simulink model "hopper_6dof_NED_v2_fluid_integration"  (R2026a)
settings: Solver=FixedStepAuto  StopTime=tgrid(end)  FixedStep=1e-3  RelTol=1e-5
InitFcn:
  | load('FuelPropsData.mat');
undefined symbols (not defined in the file): cg_init, dcg_dMfu_table, dcg_dMox_table, dI_dMfu_table, dI_dMox_table, ENGINE, engine_cg, engine_mass, fu_axial_damping_ratios, fu_lateral_damping_ratios, fu_mass_profile, fu_masses, fu_mdot_data, g, IN, K1flat, K2grid, MoI_init, mount_cg, OUT, ox_axial_damping_ratios, ox_lateral_damping_ratios, ox_mass_profile, ox_masses, ox_mdot_data, pressureLevels, r_leg, r_leg_1, r_leg_2, r_leg_3, r_leg_4, STRUCT, tank_r, TANKS, Target_Trajectory, tgrid, thrust_data, unom, uwndTable, VEH, vwndTable
libraries: fl_lib x43, nesl_utility x31, matrix_library x18, SimscapeFluids_lib x13, simulink x8, simulink_extras x7, slpidlib x7, dspindex x3, dspmtrx3 x3, sl_discontinuities x2, aerolibanim x1, commrandsrc3 x1
(part 7 of 7)

== system hopper_6dof_NED_v2_fluid_integration/Wind Forces/If Action Subsystem2 ==
  In1 : Inport
  Action Port : ActionPort  ActionPortLabel=else
  Display : Display
  Display1 : Display
  Latitude : Constant  Value=33.78
  Longitude : Constant  Value=84.40
  Month : Constant  Value=4
  Mux : Mux  Inputs=2
  Pressure (mb) : Constant  Value=1000
  Terminator : Terminator
  n-D Lookup Table : Lookup_n-D  NumberOfTableDimensions=4  BreakpointsForDimension1=1:12  BreakpointsForDimension2=pressureLevels  BreakpointsForDimension3=[32.5 35]  BreakpointsForDimension4=[82.5 85]  Table=uwndTable  ExtrapMethod=Clip  InternalRulePriority=Speed  RndMeth=Simplest
      settings: InputPortMap=u0,u1,u2,u3
  n-D Lookup Table1 : Lookup_n-D  NumberOfTableDimensions=4  BreakpointsForDimension1=1:12  BreakpointsForDimension2=pressureLevels  BreakpointsForDimension3=[32.5 35]  BreakpointsForDimension4=[82.5 85]  Table=vwndTable  InternalRulePriority=Speed  RndMeth=Simplest
      settings: InputPortMap=u0,u1,u2,u3
  Out1 : Outport
  wires:
  Month/1 -> n-D Lookup Table1/1, n-D Lookup Table/1
  Pressure (mb)/1 -> n-D Lookup Table1/2, n-D Lookup Table/2
  Latitude/1 -> n-D Lookup Table1/3, n-D Lookup Table/3
  In1/1 -> Terminator/1
  Longitude/1 -> n-D Lookup Table1/4, n-D Lookup Table/4
  n-D Lookup Table/1 -> Display/1, Mux/1
  n-D Lookup Table1/1 -> Display1/1, Mux/2
  Mux/1 -> Out1/1

== system hopper_6dof_NED_v2_fluid_integration/Fluid Network2/COPV/COPV Leakage ==
  Leak Rate : fl_lib/Gas/Elements/Flow Resistance (G)  delta_p_nominal=0.001 MPa  mdot_nominal=0.0000000001 kg/s  rho_nominal=0 kg/m^3  area=0.01 m^2  laminar_fraction=1e-3
  Mass & Energy Flow Rate Sensor (G)2 : fl_lib/Gas/Sensors/Flow Rate Sensor (G)  mass_flow_measure=true  volumetric_flow_measure=false  volumetric_flow_conditions=foundation.enum.volumetric_flow_conditions.actual  p_std=0.101325 MPa  T_std=20 degC  energy_flow_measure=true
  PS-Simulink Converter7 : nesl_utility/PS-Simulink Converter  PhysicalDomain=network_engine_domain  SubClassName=ps_output  LeftPortType=input  RightPortType=output  PseudoPeriodic=off  Frequencies=[]  VectorFormat=inherit  Unit=inherit  AffineConversion=off
  Pressurant Mass Leak Rate : Scope  Commented=on
      settings: ActiveDisplayYMinimum=-1  ActiveDisplayYMaximum=1
  Reservoir (G) : fl_lib/Gas/Elements/Reservoir (G)  pressure_input=false  pressure_spec=foundation.enum.pressure_spec.atmospheric  reservoir_pressure=0.101325 MPa  temperature_input=false  reservoir_temperature=293.15 K  area_A=0.01 m^2  input_error_spec=foundation.enum.input_range_error.warn
  Conn1 : PMIOPort  Side=Right
  wires:
  PS-Simulink Converter7/1 -> Pressurant Mass Leak Rate/1
  connections:
  Conn1/RConn1 -- Leak Rate/RConn1
  Leak Rate/LConn1 -- Mass & Energy Flow Rate Sensor (G)2/LConn1
  Mass & Energy Flow Rate Sensor (G)2/RConn1 -- Reservoir (G)/LConn1
  Mass & Energy Flow Rate Sensor (G)2/RConn2 -- PS-Simulink Converter7/LConn1

== system hopper_6dof_NED_v2_fluid_integration/Fluid Network2/Physical Combustion Chamber1/Ox Tank PT + Initial Conditions2 ==
  Initial OT Pressure : InitialCondition  Value=500
  PS-Simulink Converter3 : nesl_utility/PS-Simulink Converter  PhysicalDomain=network_engine_domain  SubClassName=ps_output  LeftPortType=input  RightPortType=output  PseudoPeriodic=off  Frequencies=[]  VectorFormat=inherit  Unit=inherit  AffineConversion=off
  Pa to psi : Gain  Gain=0.000145038
  Pressure & Temperature Sensor (TL) : fl_lib/Thermal Liquid/Sensors/Pressure & Temperature Sensor (TL)  reference=foundation.enum.MeasurementReference.absolute  pressure=true  pressure_spec=foundation.enum.PressureMeasementSpec.Gauge  temperature=false
  fuel line : PMIOPort  Side=Left
  Out1 : Outport
  wires:
  Initial OT Pressure/1 -> Out1/1
  Pa to psi/1 -> Initial OT Pressure/1
  PS-Simulink Converter3/1 -> Pa to psi/1
  connections:
  PS-Simulink Converter3/LConn1 -- Pressure & Temperature Sensor (TL)/RConn1
  Pressure & Temperature Sensor (TL)/LConn1 -- fuel line/RConn1

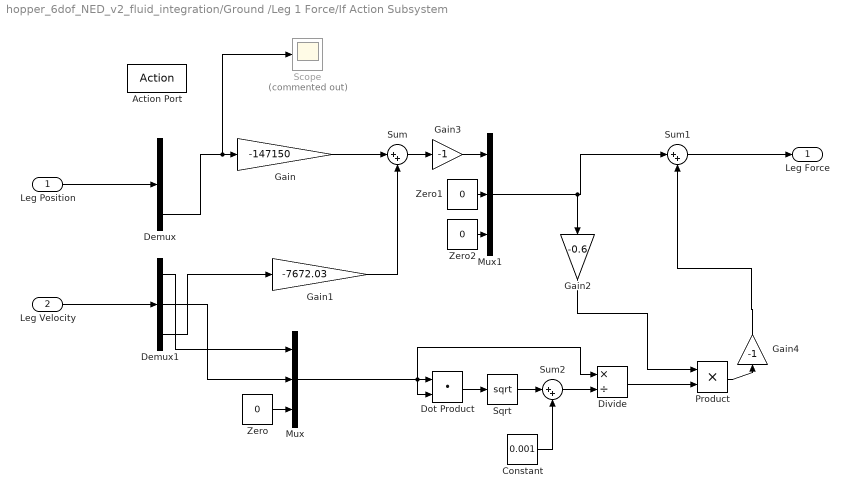
== system hopper_6dof_NED_v2_fluid_integration/Ground /Leg 1 Force/If Action Subsystem ==
  Leg Position : Inport
  Leg Velocity : Inport  Port=2
  Action Port : ActionPort  ActionPortLabel=|
      | if(u1 > -0.001 
      | )
  Constant : Constant  Value=0.001
  Demux : Demux  Outputs=3
  Demux1 : Demux  Outputs=3
  Divide : Product  Inputs=*/
  Dot Product : DotProduct  OutDataTypeStr=Inherit: Inherit via internal rule
  Gain : Gain  Gain=-147150
  Gain1 : Gain  Gain=-7672.03
  Gain2 : Gain  Gain=-0.6
  Gain3 : Gain  Gain=-1
  Gain4 : Gain  Gain=-1
  Mux : Mux  Inputs=3
  Mux1 : Mux  Inputs=3
  Product : Product
  Scope : Scope  Commented=on
      settings: ActiveDisplayYMinimum=-1  ActiveDisplayYMaximum=1  DataLoggingVariableName=ScopeData69
  Sqrt : Sqrt
  Sum : Sum  Inputs=|++
  Sum1 : Sum  Inputs=|++
  Sum2 : Sum  Inputs=|++
  Zero : Constant  Value=0  OutDataTypeStr=Inherit: Inherit via back propagation
  Zero1 : Constant  Value=0  OutDataTypeStr=Inherit: Inherit via back propagation
  Zero2 : Constant  Value=0  OutDataTypeStr=Inherit: Inherit via back propagation
  Leg Force : Outport
  wires:
  Leg Position/1 -> Demux/1
  Leg Velocity/1 -> Demux1/1
  Gain/1 -> Sum/1
  Gain1/1 -> Sum/2
  Demux1/3 -> Gain1/1
  Demux1/2 -> Mux/2
  Demux1/1 -> Mux/1
  Mux/1 -> Dot Product/2, Dot Product/1, Divide/1
  Dot Product/1 -> Sqrt/1
  Divide/1 -> Product/2
  Gain2/1 -> Product/1
  Product/1 -> Gain4/1
  Sum1/1 -> Leg Force/1
  Sqrt/1 -> Sum2/1
  Sum2/1 -> Divide/2
  Constant/1 -> Sum2/2
  Sum/1 -> Gain3/1
  Zero1/1 -> Mux1/2
  Zero2/1 -> Mux1/3
  Mux1/1 -> Sum1/1, Gain2/1
  Demux/3 -> Scope/1, Gain/1
  Zero/1 -> Mux/3
  Gain3/1 -> Mux1/1
  Gain4/1 -> Sum1/2

== system hopper_6dof_NED_v2_fluid_integration/Ground /Leg 1 Force/If Action Subsystem1 ==
  Action Port : ActionPort  ActionPortLabel=else
  Constant : Constant  Value=[0 0 0]
  Out1 : Outport
  wires:
  Constant/1 -> Out1/1

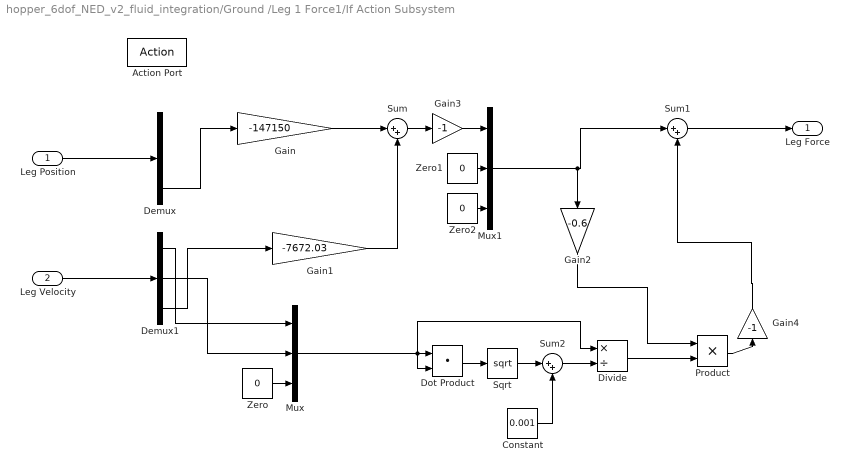
== system hopper_6dof_NED_v2_fluid_integration/Ground /Leg 1 Force1/If Action Subsystem ==
  Leg Position : Inport
  Leg Velocity : Inport  Port=2
  Action Port : ActionPort  ActionPortLabel=|
      | if(u1 > -0.001 
      | )
  Constant : Constant  Value=0.001
  Demux : Demux  Outputs=3
  Demux1 : Demux  Outputs=3
  Divide : Product  Inputs=*/
  Dot Product : DotProduct  OutDataTypeStr=Inherit: Inherit via internal rule
  Gain : Gain  Gain=-147150
  Gain1 : Gain  Gain=-7672.03
  Gain2 : Gain  Gain=-0.6
  Gain3 : Gain  Gain=-1
  Gain4 : Gain  Gain=-1
  Mux : Mux  Inputs=3
  Mux1 : Mux  Inputs=3
  Product : Product
  Sqrt : Sqrt
  Sum : Sum  Inputs=|++
  Sum1 : Sum  Inputs=|++
  Sum2 : Sum  Inputs=|++
  Zero : Constant  Value=0  OutDataTypeStr=Inherit: Inherit via back propagation
  Zero1 : Constant  Value=0  OutDataTypeStr=Inherit: Inherit via back propagation
  Zero2 : Constant  Value=0  OutDataTypeStr=Inherit: Inherit via back propagation
  Leg Force : Outport
  wires:
  Leg Position/1 -> Demux/1
  Leg Velocity/1 -> Demux1/1
  Gain/1 -> Sum/1
  Gain1/1 -> Sum/2
  Demux1/3 -> Gain1/1
  Demux1/2 -> Mux/2
  Demux1/1 -> Mux/1
  Mux/1 -> Dot Product/2, Dot Product/1, Divide/1
  Dot Product/1 -> Sqrt/1
  Divide/1 -> Product/2
  Gain2/1 -> Product/1
  Product/1 -> Gain4/1
  Sum1/1 -> Leg Force/1
  Sqrt/1 -> Sum2/1
  Sum2/1 -> Divide/2
  Constant/1 -> Sum2/2
  Sum/1 -> Gain3/1
  Zero1/1 -> Mux1/2
  Zero2/1 -> Mux1/3
  Mux1/1 -> Sum1/1, Gain2/1
  Demux/3 -> Gain/1
  Zero/1 -> Mux/3
  Gain3/1 -> Mux1/1
  Gain4/1 -> Sum1/2

== system hopper_6dof_NED_v2_fluid_integration/Ground /Leg 1 Force1/If Action Subsystem1 ==
  Action Port : ActionPort  ActionPortLabel=else
  Constant : Constant  Value=[0 0 0]
  Out1 : Outport
  wires:
  Constant/1 -> Out1/1

== system hopper_6dof_NED_v2_fluid_integration/Ground /Leg 1 Force2/If Action Subsystem ==
  Leg Position : Inport
  Leg Velocity : Inport  Port=2
  Action Port : ActionPort  ActionPortLabel=|
      | if(u1 > -0.001 
      | )
  Constant : Constant  Value=0.001
  Demux : Demux  Outputs=3
  Demux1 : Demux  Outputs=3
  Divide : Product  Inputs=*/
  Dot Product : DotProduct  OutDataTypeStr=Inherit: Inherit via internal rule
  Gain : Gain  Gain=-147150
  Gain1 : Gain  Gain=-7672.03
  Gain2 : Gain  Gain=-0.6
  Gain3 : Gain  Gain=-1
  Gain4 : Gain  Gain=-1
  Mux : Mux  Inputs=3
  Mux1 : Mux  Inputs=3
  Product : Product
  Sqrt : Sqrt
  Sum : Sum  Inputs=|++
  Sum1 : Sum  Inputs=|++
  Sum2 : Sum  Inputs=|++
  Zero : Constant  Value=0  OutDataTypeStr=Inherit: Inherit via back propagation
  Zero1 : Constant  Value=0  OutDataTypeStr=Inherit: Inherit via back propagation
  Zero2 : Constant  Value=0  OutDataTypeStr=Inherit: Inherit via back propagation
  Leg Force : Outport
  wires:
  Leg Position/1 -> Demux/1
  Leg Velocity/1 -> Demux1/1
  Gain/1 -> Sum/1
  Gain1/1 -> Sum/2
  Demux1/3 -> Gain1/1
  Demux1/2 -> Mux/2
  Demux1/1 -> Mux/1
  Mux/1 -> Dot Product/2, Dot Product/1, Divide/1
  Dot Product/1 -> Sqrt/1
  Divide/1 -> Product/2
  Gain2/1 -> Product/1
  Product/1 -> Gain4/1
  Sum1/1 -> Leg Force/1
  Sqrt/1 -> Sum2/1
  Sum2/1 -> Divide/2
  Constant/1 -> Sum2/2
  Sum/1 -> Gain3/1
  Zero1/1 -> Mux1/2
  Zero2/1 -> Mux1/3
  Mux1/1 -> Sum1/1, Gain2/1
  Demux/3 -> Gain/1
  Zero/1 -> Mux/3
  Gain3/1 -> Mux1/1
  Gain4/1 -> Sum1/2

== system hopper_6dof_NED_v2_fluid_integration/Ground /Leg 1 Force2/If Action Subsystem1 ==
  Action Port : ActionPort  ActionPortLabel=else
  Constant : Constant  Value=[0 0 0]
  Out1 : Outport
  wires:
  Constant/1 -> Out1/1

== system hopper_6dof_NED_v2_fluid_integration/Ground /Leg 1 Force3/If Action Subsystem ==
  Leg Position : Inport
  Leg Velocity : Inport  Port=2
  Action Port : ActionPort  ActionPortLabel=|
      | if(u1 > -0.001 
      | )
  Constant : Constant  Value=0.001
  Demux : Demux  Outputs=3
  Demux1 : Demux  Outputs=3
  Divide : Product  Inputs=*/
  Dot Product : DotProduct  OutDataTypeStr=Inherit: Inherit via internal rule
  Gain : Gain  Gain=-147150
  Gain1 : Gain  Gain=-7672.03
  Gain2 : Gain  Gain=-0.6
  Gain3 : Gain  Gain=-1
  Gain4 : Gain  Gain=-1
  Mux : Mux  Inputs=3
  Mux1 : Mux  Inputs=3
  Product : Product
  Sqrt : Sqrt
  Sum : Sum  Inputs=|++
  Sum1 : Sum  Inputs=|++
  Sum2 : Sum  Inputs=|++
  Zero : Constant  Value=0  OutDataTypeStr=Inherit: Inherit via back propagation
  Zero1 : Constant  Value=0  OutDataTypeStr=Inherit: Inherit via back propagation
  Zero2 : Constant  Value=0  OutDataTypeStr=Inherit: Inherit via back propagation
  Leg Force : Outport
  wires:
  Leg Position/1 -> Demux/1
  Leg Velocity/1 -> Demux1/1
  Gain/1 -> Sum/1
  Gain1/1 -> Sum/2
  Demux1/3 -> Gain1/1
  Demux1/2 -> Mux/2
  Demux1/1 -> Mux/1
  Mux/1 -> Dot Product/2, Dot Product/1, Divide/1
  Dot Product/1 -> Sqrt/1
  Divide/1 -> Product/2
  Gain2/1 -> Product/1
  Product/1 -> Gain4/1
  Sum1/1 -> Leg Force/1
  Sqrt/1 -> Sum2/1
  Sum2/1 -> Divide/2
  Constant/1 -> Sum2/2
  Sum/1 -> Gain3/1
  Zero1/1 -> Mux1/2
  Zero2/1 -> Mux1/3
  Mux1/1 -> Sum1/1, Gain2/1
  Demux/3 -> Gain/1
  Zero/1 -> Mux/3
  Gain3/1 -> Mux1/1
  Gain4/1 -> Sum1/2

== system hopper_6dof_NED_v2_fluid_integration/Ground /Leg 1 Force3/If Action Subsystem1 ==
  Action Port : ActionPort  ActionPortLabel=else
  Constant : Constant  Value=[0 0 0]
  Out1 : Outport
  wires:
  Constant/1 -> Out1/1

== matlab function hopper_6dof_NED_v2_fluid_integration/Slosh/Oxidizer Yaw Force/MATLAB Function ==
  data: ox_yaw_accel input; accel_term output; ox_lateral_pendulum_l input
function accel_term = fcn(ox_yaw_accel, ox_lateral_pendulum_l)

accel_term = -ox_yaw_accel / ox_lateral_pendulum_l;

end

== matlab function hopper_6dof_NED_v2_fluid_integration/Slosh/Oxidizer Yaw Force/MATLAB Function1 ==
  data: ox_yaw_phi input; ang_term output; ox_lateral_natural_freq input
function ang_term = fcn(ox_yaw_phi, ox_lateral_natural_freq)

ang_term = -ox_lateral_natural_freq^2 * ox_yaw_phi;

end

== matlab function hopper_6dof_NED_v2_fluid_integration/Slosh/Oxidizer Yaw Force/MATLAB Function2 ==
  data: ox_yaw_phi_dot input; velo_term output; ox_lateral_natural_freq input; ox_lateral_damping input
function velo_term = fcn(ox_yaw_phi_dot, ox_lateral_natural_freq,ox_lateral_damping)

velo_term = -2 * ox_lateral_damping * ox_lateral_natural_freq * ox_yaw_phi_dot;
end

== matlab function hopper_6dof_NED_v2_fluid_integration/Slosh/Oxidizer Yaw Force/MATLAB Function3 ==
  data: ox_yaw_phi_ddot input; ox_yaw_f output; ox_lateral_slosh_mass input; ox_lateral_pendulum_l input
function ox_yaw_f = fcn(ox_yaw_phi_ddot, ox_lateral_slosh_mass, ox_lateral_pendulum_l)
% Force of the pendulum on the tank, beyond the rigid propellant already in
% the vehicle mass: -m1 * y_ddot, y = l*phi the body-frame bob displacement
% (phi_ddot = -a/l - w^2 phi - 2 zeta w phi_dot). Sign was +m1*y_ddot,
% which added m1 to the lateral inertia instead of removing it.
ox_yaw_f = -ox_lateral_slosh_mass * ox_lateral_pendulum_l * ox_yaw_phi_ddot;
end

== matlab function hopper_6dof_NED_v2_fluid_integration/Slosh/Oxidizer Axial Force/MATLAB Function ==
  data: ox_axial_accel input; accel_term output; ox_axial_pendulum_l input
function accel_term = fcn(ox_axial_accel, ox_axial_pendulum_l)

accel_term = -ox_axial_accel / ox_axial_pendulum_l;

end

== matlab function hopper_6dof_NED_v2_fluid_integration/Slosh/Oxidizer Axial Force/MATLAB Function1 ==
  data: ox_axial_phi input; ang_term output; ox_axial_natural_freq input
function ang_term = fcn(ox_axial_phi, ox_axial_natural_freq)

ang_term = -ox_axial_natural_freq^2 * ox_axial_phi;

end

== matlab function hopper_6dof_NED_v2_fluid_integration/Slosh/Oxidizer Axial Force/MATLAB Function2 ==
  data: ox_axial_phi_dot input; velo_term output; ox_axial_natural_freq input; ox_axial_damping input
function velo_term = fcn(ox_axial_phi_dot, ox_axial_natural_freq,ox_axial_damping)

velo_term = -2 * ox_axial_damping * ox_axial_natural_freq * ox_axial_phi_dot;
end

== matlab function hopper_6dof_NED_v2_fluid_integration/Slosh/Oxidizer Axial Force/MATLAB Function3 ==
  data: ox_axial_phi_ddot input; ox_axial_f output; ox_axial_slosh_mass input; ox_axial_pendulum_l input
function ox_axial_f = fcn(ox_axial_phi_ddot, ox_axial_slosh_mass, ox_axial_pendulum_l)
% Force of the pendulum on the tank, beyond the rigid propellant already in
% the vehicle mass: -m1 * y_ddot, y = l*phi the body-frame bob displacement
% (phi_ddot = -a/l - w^2 phi - 2 zeta w phi_dot). Sign was +m1*y_ddot,
% which added m1 to the lateral inertia instead of removing it.
ox_axial_f = -ox_axial_slosh_mass * ox_axial_pendulum_l * ox_axial_phi_ddot;
end

== matlab function hopper_6dof_NED_v2_fluid_integration/Slosh/Fuel Axial Force/MATLAB Function ==
  data: fu_axial_accel input; accel_term output; fu_axial_pendulum_l input
function accel_term = fcn(fu_axial_accel, fu_axial_pendulum_l)

accel_term = -fu_axial_accel / fu_axial_pendulum_l;

end

== matlab function hopper_6dof_NED_v2_fluid_integration/Slosh/Fuel Axial Force/MATLAB Function1 ==
  data: fu_axial_phi input; ang_term output; fu_axial_natural_freq input
function ang_term = fcn(fu_axial_phi, fu_axial_natural_freq)

ang_term = -fu_axial_natural_freq^2 * fu_axial_phi;

end

== matlab function hopper_6dof_NED_v2_fluid_integration/Slosh/Fuel Axial Force/MATLAB Function2 ==
  data: fu_axial_phi_dot input; velo_term output; fu_axial_natural_freq input; fu_axial_damping input
function velo_term = fcn(fu_axial_phi_dot, fu_axial_natural_freq,fu_axial_damping)

velo_term = -2 * fu_axial_damping * fu_axial_natural_freq * fu_axial_phi_dot;
end

== matlab function hopper_6dof_NED_v2_fluid_integration/Slosh/Fuel Axial Force/MATLAB Function3 ==
  data: fu_axial_phi_ddot input; fu_axial_f output; fu_axial_slosh_mass input; fu_axial_pendulum_l input
function fu_axial_f = fcn(fu_axial_phi_ddot, fu_axial_slosh_mass, fu_axial_pendulum_l)
% Force of the pendulum on the tank, beyond the rigid propellant already in
% the vehicle mass: -m1 * y_ddot, y = l*phi the body-frame bob displacement
% (phi_ddot = -a/l - w^2 phi - 2 zeta w phi_dot). Sign was +m1*y_ddot,
% which added m1 to the lateral inertia instead of removing it.
fu_axial_f = -fu_axial_slosh_mass * fu_axial_pendulum_l * fu_axial_phi_ddot;
end

== matlab function hopper_6dof_NED_v2_fluid_integration/Slosh/Fuel Yaw Force/MATLAB Function ==
  data: fu_pitch_accel input; accel_term output; fu_lateral_pendulum_l input
function accel_term = fcn(fu_pitch_accel, fu_lateral_pendulum_l)

accel_term = -fu_pitch_accel / fu_lateral_pendulum_l;

end

== matlab function hopper_6dof_NED_v2_fluid_integration/Slosh/Fuel Yaw Force/MATLAB Function1 ==
  data: fu_pitch_phi input; ang_term output; fu_lateral_natural_freq input
function ang_term = fcn(fu_pitch_phi, fu_lateral_natural_freq)

ang_term = -fu_lateral_natural_freq^2 * fu_pitch_phi;

end

== matlab function hopper_6dof_NED_v2_fluid_integration/Slosh/Fuel Yaw Force/MATLAB Function2 ==
  data: fu_pitch_phi_dot input; velo_term output; fu_lateral_natural_freq input; fu_lateral_damping input
function velo_term = fcn(fu_pitch_phi_dot, fu_lateral_natural_freq,fu_lateral_damping)

velo_term = -2 * fu_lateral_damping * fu_lateral_natural_freq * fu_pitch_phi_dot;
end

== matlab function hopper_6dof_NED_v2_fluid_integration/Slosh/Fuel Yaw Force/MATLAB Function3 ==
  data: fu_pitch_phi_ddot input; fu_pitch_f output; fu_lateral_slosh_mass input; fu_lateral_pendulum_l input
function fu_pitch_f = fcn(fu_pitch_phi_ddot, fu_lateral_slosh_mass, fu_lateral_pendulum_l)
% Force of the pendulum on the tank, beyond the rigid propellant already in
% the vehicle mass: -m1 * y_ddot, y = l*phi the body-frame bob displacement
% (phi_ddot = -a/l - w^2 phi - 2 zeta w phi_dot). Sign was +m1*y_ddot,
% which added m1 to the lateral inertia instead of removing it.
fu_pitch_f = -fu_lateral_slosh_mass * fu_lateral_pendulum_l * fu_pitch_phi_ddot;
end

== matlab function hopper_6dof_NED_v2_fluid_integration/Slosh/Fuel Pitch Force/MATLAB Function ==
  data: fu_yaw_accel input; accel_term output; fu_lateral_pendulum_l input
function accel_term = fcn(fu_yaw_accel, fu_lateral_pendulum_l)

accel_term = -fu_yaw_accel / fu_lateral_pendulum_l;

end

== matlab function hopper_6dof_NED_v2_fluid_integration/Slosh/MATLAB Function ==
  data: ox_lateral_natural_freq output; ox_axial_natural_freq output; ox_mass input; ox_lateral_slosh_mass output; ox_axial_slosh_mass output; ox_lateral_pendulum_l output; ox_aeff input; ox_axial_pendulum_l output; ox_lateral_damping output; ox_axial_damping output; tank_r input; ox_lateral_damping input; ox_axial_damping input
function [ox_lateral_natural_freq, ox_axial_natural_freq, ox_lateral_slosh_mass,ox_axial_slosh_mass, ox_lateral_pendulum_l, ox_axial_pendulum_l, ox_lateral_damping, ox_axial_damping]  = slosh_parameters(ox_mass, ox_aeff, tank_r, ox_lateral_damping, ox_axial_damping)

% Flat-bottomed cylindrical tank, linear slosh (NASA SP-106 / Dodge 2000;
% lateral values checked against SLOSH-ML, lgst-lab/slosh_ml).
zeta = 1.841;    % 1st root of J1' (1st lateral mode)
eps01 = 3.8317;  % 1st root of J1 (1st axisymmetric mode)
ox_density = 1141;   % kg/m^3
geff = norm(ox_aeff) + 0.001;

if ox_mass > 0.001
   h_ox_fluid = (ox_mass / ox_density) / (pi * tank_r^2);

   % Lateral mode: omega^2 = (g*xi/R) * tanh(xi*h/R)
    ox_lateral_natural_freq = sqrt(zeta * geff / tank_r * tanh(zeta * h_ox_fluid / tank_r));
    ox_lateral_slosh_mass = ox_mass * (2 * tank_r * tanh(zeta * h_ox_fluid / tank_r)) / (zeta * (zeta^2 - 1) * h_ox_fluid);
    ox_lateral_pendulum_l = tank_r / (zeta * tanh(zeta * h_ox_fluid / tank_r));   % = geff / omega^2

    % Axisymmetric (m = 0) mode: omega^2 = (g*eps01/R) * tanh(eps01*h/R).
    % Volume is conserved and the mode is axisymmetric, so to first order
    % it puts no net force or moment on the tank: its equivalent mechanical
    % mass is zero. The oscillator is kept (frequency/damping) but couples
    % no force or roll torque into the vehicle.
    ox_axial_natural_freq = sqrt(eps01 * geff / tank_r * tanh(eps01 * h_ox_fluid / tank_r));
    ox_axial_slosh_mass = 0;
    ox_axial_pendulum_l = geff / ox_axial_natural_freq^2;
else
   h_ox_fluid = 0;
   ox_lateral_natural_freq = 0;
   ox_axial_natural_freq = 0;
   ox_lateral_slosh_mass = 0;
   ox_axial_slosh_mass = 0;
   ox_lateral_pendulum_l = 1;
   ox_axial_pendulum_l = 1;
end

end

== matlab function hopper_6dof_NED_v2_fluid_integration/Slosh/Fuel Pitch Force/MATLAB Function1 ==
  data: fu_yaw_phi input; ang_term output; fu_lateral_natural_freq input
function ang_term = fcn(fu_yaw_phi, fu_lateral_natural_freq)

ang_term = -fu_lateral_natural_freq^2 * fu_yaw_phi;

end

== matlab function hopper_6dof_NED_v2_fluid_integration/Slosh/Fuel Pitch Force/MATLAB Function2 ==
  data: fu_yaw_phi_dot input; velo_term output; fu_lateral_natural_freq input; fu_lateral_damping input
function velo_term = fcn(fu_yaw_phi_dot, fu_lateral_natural_freq, fu_lateral_damping)

velo_term = -2 * fu_lateral_damping * fu_lateral_natural_freq * fu_yaw_phi_dot;
end

== matlab function hopper_6dof_NED_v2_fluid_integration/Slosh/Fuel Pitch Force/MATLAB Function3 ==
  data: fu_yaw_phi_ddot input; fu_yaw_f output; fu_lateral_slosh_mass input; fu_lateral_pendulum_l input
function fu_yaw_f = fcn(fu_yaw_phi_ddot, fu_lateral_slosh_mass, fu_lateral_pendulum_l)
% Force of the pendulum on the tank, beyond the rigid propellant already in
% the vehicle mass: -m1 * y_ddot, y = l*phi the body-frame bob displacement
% (phi_ddot = -a/l - w^2 phi - 2 zeta w phi_dot). Sign was +m1*y_ddot,
% which added m1 to the lateral inertia instead of removing it.
fu_yaw_f = -fu_lateral_slosh_mass * fu_lateral_pendulum_l * fu_yaw_phi_ddot;
end

== matlab function hopper_6dof_NED_v2_fluid_integration/CG // MOI Script v3/MATLAB Function ==
  data: r_ox input; I_m_ox output
function I_m_ox = fcn(r_ox)
% Slosh point-mass inertia contribution. The base MOI (cg_moi_init /
% dI_dMox LUT) already carries all the propellant as a rigid body, and
% the slosh pendulum dynamics reach the vehicle through Slosh_F / Slosh_M,
% so adding the slosh masses again here double counts them (and r_ox is
% measured from the vehicle datum, not the CG). Contribution removed;
% output kept so the block interface is unchanged.
% (Previous parallel-axis tensor also had sign errors in its products
% of inertia and was not symmetric.)
I_m_ox = zeros(3) * r_ox(1);

== matlab function hopper_6dof_NED_v2_fluid_integration/CG // MOI Script v3/MATLAB Function1 ==
  data: r_fu input; I_m_fu output
function I_m_fu = fcn(r_fu)
% Slosh point-mass inertia contribution. The base MOI (cg_moi_init /
% dI_dMfu LUT) already carries all the propellant as a rigid body, and
% the slosh pendulum dynamics reach the vehicle through Slosh_F / Slosh_M,
% so adding the slosh masses again here double counts them (and r_fu is
% measured from the vehicle datum, not the CG). Contribution removed;
% output kept so the block interface is unchanged.
% (Previous parallel-axis tensor also had sign errors in its products
% of inertia and was not symmetric.)
I_m_fu = zeros(3) * r_fu(1);

== matlab function hopper_6dof_NED_v2_fluid_integration/Slosh/Oxidizer Axial Force/MATLAB Function4 ==
  data: x_omega_dot input; x_slosh_torque output; ox_axial_slosh_mass input; ox_axial_pendulum_l input; slosh_angular_accel input
function x_slosh_torque = fcn(x_omega_dot, ox_axial_slosh_mass, ox_axial_pendulum_l, slosh_angular_accel)
% Per-pendulum torque removed. A pendulum analog (SP-106, Dodge 2000,
% SLOSH-ML) is a point mass on a frictionless hinge: it has no rotational
% inertia of its own and transmits no moment through the hinge. The old
% -m*l^2*(omega_dot - phi_ddot) term added a fictitious inertia m*l^2 and a
% hinge moment. The liquid rigid-body inertia (the analog's I0) is carried
% by the CG/MOI tables. Inputs kept for the
% subsystem interface.
x_slosh_torque = 0 * x_omega_dot;
end

== matlab function hopper_6dof_NED_v2_fluid_integration/Slosh/Fuel Axial Force/MATLAB Function4 ==
  data: x_omega_dot input; x_slosh_torque output; fu_axial_slosh_mass input; fu_axial_pendulum_l input; slosh_angular_accel input
function x_slosh_torque = fcn(x_omega_dot, fu_axial_slosh_mass, fu_axial_pendulum_l, slosh_angular_accel)
% Per-pendulum torque removed. A pendulum analog (SP-106, Dodge 2000,
% SLOSH-ML) is a point mass on a frictionless hinge: it has no rotational
% inertia of its own and transmits no moment through the hinge. The old
% -m*l^2*(omega_dot - phi_ddot) term added a fictitious inertia m*l^2 and a
% hinge moment. The liquid rigid-body inertia (the analog's I0) is carried
% by the CG/MOI tables. Inputs kept for the
% subsystem interface.
x_slosh_torque = 0 * x_omega_dot;
end

== matlab function hopper_6dof_NED_v2_fluid_integration/Slosh/Oxidizer Yaw Force/MATLAB Function4 ==
  data: y_omega_dot input; y_slosh_torque output; ox_lateral_slosh_mass input; ox_lateral_pendulum_l input; slosh_angular_accel input
function y_slosh_torque = fcn(y_omega_dot, ox_lateral_slosh_mass, ox_lateral_pendulum_l, slosh_angular_accel)
% Per-pendulum torque removed. A pendulum analog (SP-106, Dodge 2000,
% SLOSH-ML) is a point mass on a frictionless hinge: it has no rotational
% inertia of its own and transmits no moment through the hinge. The old
% -m*l^2*(omega_dot - phi_ddot) term added a fictitious inertia m*l^2 and a
% hinge moment. The liquid rigid-body inertia (the analog's I0) is carried
% by the CG/MOI tables. Inputs kept for the
% subsystem interface.
y_slosh_torque = 0 * y_omega_dot;
end

== matlab function hopper_6dof_NED_v2_fluid_integration/Slosh/Fuel Yaw Force/MATLAB Function4 ==
  data: y_omega_dot input; y_slosh_torque output; fu_lateral_slosh_mass input; fu_lateral_pendulum_l input; slosh_angular_accel input
function y_slosh_torque = fcn(y_omega_dot, fu_lateral_slosh_mass, fu_lateral_pendulum_l, slosh_angular_accel)
% Per-pendulum torque removed. A pendulum analog (SP-106, Dodge 2000,
% SLOSH-ML) is a point mass on a frictionless hinge: it has no rotational
% inertia of its own and transmits no moment through the hinge. The old
% -m*l^2*(omega_dot - phi_ddot) term added a fictitious inertia m*l^2 and a
% hinge moment. The liquid rigid-body inertia (the analog's I0) is carried
% by the CG/MOI tables. Inputs kept for the
% subsystem interface.
y_slosh_torque = 0 * y_omega_dot;
end

== matlab function hopper_6dof_NED_v2_fluid_integration/Slosh/Oxidizer Pitch Force/MATLAB Function4 ==
  data: z_omega_dot input; z_slosh_torque output; ox_lateral_slosh_mass input; ox_lateral_pendulum_l input; slosh_angular_accel input
function z_slosh_torque = fcn(z_omega_dot, ox_lateral_slosh_mass, ox_lateral_pendulum_l, slosh_angular_accel)
% Per-pendulum torque removed. A pendulum analog (SP-106, Dodge 2000,
% SLOSH-ML) is a point mass on a frictionless hinge: it has no rotational
% inertia of its own and transmits no moment through the hinge. The old
% -m*l^2*(omega_dot - phi_ddot) term added a fictitious inertia m*l^2 and a
% hinge moment. The liquid rigid-body inertia (the analog's I0) is carried
% by the CG/MOI tables. Inputs kept for the
% subsystem interface.
z_slosh_torque = 0 * z_omega_dot;
end

== matlab function hopper_6dof_NED_v2_fluid_integration/Slosh/Fuel Pitch Force/MATLAB Function4 ==
  data: z_omega_dot input; z_slosh_torque output; fu_lateral_slosh_mass input; fu_lateral_pendulum_l input; slosh_angular_accel input
function z_slosh_torque = fcn(z_omega_dot, fu_lateral_slosh_mass, fu_lateral_pendulum_l, slosh_angular_accel)
% Per-pendulum torque removed. A pendulum analog (SP-106, Dodge 2000,
% SLOSH-ML) is a point mass on a frictionless hinge: it has no rotational
% inertia of its own and transmits no moment through the hinge. The old
% -m*l^2*(omega_dot - phi_ddot) term added a fictitious inertia m*l^2 and a
% hinge moment. The liquid rigid-body inertia (the analog's I0) is carried
% by the CG/MOI tables. Inputs kept for the
% subsystem interface.
z_slosh_torque = 0 * z_omega_dot;
end

== matlab function hopper_6dof_NED_v2_fluid_integration/CG // MOI Script v3/MATLAB Function2 ==
  data: delta_y input; rot_mat output; delta_z input
function rot_mat = fcn(delta_y, delta_z)

rot_mat = [0 -delta_z delta_y;
           delta_z 0 0;
           -delta_y 0 0];

== matlab function hopper_6dof_NED_v2_fluid_integration/Slosh/Ox Slosh Mass Location ==
  data: r_floor input; r_bob output; ox_mass input; tank_r input
function r_bob = fcn(r_floor, ox_mass, tank_r)
% Rest position of the 1st lateral pendulum bob (= spring-mass location),
% flat-bottom cylinder, NASA SP-106 / Dodge 2000:
%   H1 = h - (2R/xi) tanh(xi h / 2R)  above the tank floor,
%   hinge = H1 + L1,  L1 = R / (xi tanh(xi h / R)).
% Matches SLOSH-ML (validation/slosh_ml/compareSloshML.m) to < 2 mm.
% The slosh force is applied here, not at the hinge: the propellant
% (bob included) is already a rigid body in the CG/MOI tables, so the
% pendulum correction is -m1*y_ddot at the bob rest point plus the
% offset moment -m1*y x f (Slosh offset moment blocks); together these
% equal the rod force acting at the hinge.
% r_floor is in the Slosh frame (datum x negated).
xi = 1.841;
ox_density = 1141;   % kg/m^3
h = (ox_mass / ox_density) / (pi * tank_r^2);
H1 = h - (2 * tank_r / xi) * tanh(xi * h / (2 * tank_r));
r_bob = r_floor;
r_bob(1) = r_floor(1) - H1;

== matlab function hopper_6dof_NED_v2_fluid_integration/Slosh/Fu Slosh Mass Location ==
  data: r_floor input; r_bob output; fu_mass input; tank_r input
function r_bob = fcn(r_floor, fu_mass, tank_r)
% Rest position of the 1st lateral pendulum bob (= spring-mass location),
% flat-bottom cylinder, NASA SP-106 / Dodge 2000:
%   H1 = h - (2R/xi) tanh(xi h / 2R)  above the tank floor,
%   hinge = H1 + L1,  L1 = R / (xi tanh(xi h / R)).
% Matches SLOSH-ML (validation/slosh_ml/compareSloshML.m) to < 2 mm.
% The slosh force is applied here, not at the hinge: the propellant
% (bob included) is already a rigid body in the CG/MOI tables, so the
% pendulum correction is -m1*y_ddot at the bob rest point plus the
% offset moment -m1*y x f (Slosh offset moment blocks); together these
% equal the rod force acting at the hinge.
% r_floor is in the Slosh frame (datum x negated).
xi = 1.841;
fu_density = 800;   % kg/m^3
h = (fu_mass / fu_density) / (pi * tank_r^2);
H1 = h - (2 * tank_r / xi) * tanh(xi * h / (2 * tank_r));
r_bob = r_floor;
r_bob(1) = r_floor(1) - H1;

== matlab function hopper_6dof_NED_v2_fluid_integration/Slosh/Ox Slosh Offset Moment ==
  data: ox_slosh_pos input; M output; ox_slosh_mass input; ox_a_eff input
function M = fcn(ox_slosh_pos, ox_slosh_mass, ox_a_eff)
% Moment about the CG from the slosh mass displaced by y from its rest
% point, under the specific force f at the tank: -m1 * y x f. With the
% -m1*y_ddot force at the rest point this is the first-order pendulum
% load (rod force at the hinge). Replaces the slosh CG shift in
% CG // MOI Script v3, which divided by the propellant mass instead of
% the vehicle mass, had the lateral sign reversed, and was delayed.
M = reshape(-cross(ox_slosh_mass(:) .* ox_slosh_pos(:), ox_a_eff(:)), size(ox_a_eff));

== matlab function hopper_6dof_NED_v2_fluid_integration/Slosh/Fu Slosh Offset Moment ==
  data: fu_slosh_pos input; M output; fu_slosh_mass input; fu_a_eff input
function M = fcn(fu_slosh_pos, fu_slosh_mass, fu_a_eff)
% Moment about the CG from the slosh mass displaced by y from its rest
% point, under the specific force f at the tank: -m1 * y x f. With the
% -m1*y_ddot force at the rest point this is the first-order pendulum
% load (rod force at the hinge). Replaces the slosh CG shift in
% CG // MOI Script v3, which divided by the propellant mass instead of
% the vehicle mass, had the lateral sign reversed, and was delayed.
M = reshape(-cross(fu_slosh_mass(:) .* fu_slosh_pos(:), fu_a_eff(:)), size(fu_a_eff));

== matlab function hopper_6dof_NED_v2_fluid_integration/CG // MOI Script v3/Slosh Diagnostics ==
  data: cg input; cg_with_slosh output; MOI input; ox_slosh_pos input; fu_slosh_pos input; ox_slosh_mass input; fu_slosh_mass input; m_ox input; m_fu input; M input; r_ox_tank input; r_fu_tank input; tank_r input; MOI_with_slosh output
function [cg_with_slosh, MOI_with_slosh] = fcn(cg, MOI, ox_slosh_pos, fu_slosh_pos, ox_slosh_mass, fu_slosh_mass, m_ox, m_fu, M, r_ox_tank, r_fu_tank, tank_r)
% DIAGNOSTIC ONLY: vehicle CG and inertia including the lateral slosh-mass
% displacement. Not fed back to the dynamics: the Slosh subsystem already
% applies the slosh motion as a force at the slosh-mass rest point plus an
% explicit offset moment (-m1*y x f), which is the dynamic effect of this CG
% shift. Feeding these outputs back would
% count it twice.
%
% Frame: same as the cg output (x = axial position above the datum,
% y/z lateral). Slosh positions are the bob displacements from rest (y, z
% used; the axial mode has zero mass). Rest heights above the tank floor:
% H1 = h - (2R/xi) tanh(xi h / 2R) (SP-106, flat-bottom cylinder).
xi = 1.841;
R  = tank_r;
cg = cg(:);
I0 = reshape(MOI, 3, 3);

h_ox = m_ox / (1141 * pi * R^2);
h_fu = m_fu / (800  * pi * R^2);
r1_ox = [r_ox_tank(1) + h_ox - (2*R/xi) * tanh(xi*h_ox/(2*R)); 0; 0];
r1_fu = [r_fu_tank(1) + h_fu - (2*R/xi) * tanh(xi*h_fu/(2*R)); 0; 0];
d_ox = [0; ox_slosh_pos(2); ox_slosh_pos(3)];
d_fu = [0; fu_slosh_pos(2); fu_slosh_pos(3)];
m1_ox = ox_slosh_mass(2);
m1_fu = fu_slosh_mass(2);

shift = (m1_ox * d_ox + m1_fu * d_fu) / M;
cg_with_slosh = cg + shift;

% move each slosh mass from rest to displaced (about the rigid cg), then
% transfer the whole vehicle to the shifted cg
MOI_with_slosh = I0 ...
    + m1_ox * (pa(r1_ox + d_ox - cg) - pa(r1_ox - cg)) ...
    + m1_fu * (pa(r1_fu + d_fu - cg) - pa(r1_fu - cg)) ...
    - M * pa(shift);
end

function J = pa(v)
J = (v' * v) * eye(3) - v * v';
end

== matlab function hopper_6dof_NED_v2_fluid_integration/Fluid Network2/Fuel Throttle Valve Controller/Feed Forward ==
  data: mdot input; theta output; ptank input; pset input; rho input; CdA output
function [theta, CdA] = feed_forward(mdot,ptank,pset,rho)

dp = max(ptank - pset, 1e-6); % divide by zero erro

rho = max(rho, 1e-6);
CdA = mdot / sqrt(2*dp*rho);

CdA = max(CdA, 1e-7); % divide by zero error
Cv_vector = [1e-8, 0.01, 0.06, 0.21, 0.46, 0.83, 1.35, 2.04, 2.93];
CdA_vector = Cv_vector ./ 37.97;
theta_vector = 0.9.*[20,30,40,50,60,70,80,90,100];

theta = interp1(CdA_vector, theta_vector, CdA);
theta = min(theta, 90);
theta = max(theta, 0);
end

== matlab function hopper_6dof_NED_v2_fluid_integration/Fluid Network2/Fuel Throttle Valve Controller/MATLAB Function5 ==
  data: time input; rate_limit_up output; rate_limit_down output
function [rate_limit_up, rate_limit_down] = fcn(time)
if time < 0.5
    rate_limit_up = 1350;
else
    rate_limit_up = 40;
end
rate_limit_down = -rate_limit_up;

== matlab function hopper_6dof_NED_v2_fluid_integration/MATLAB Function ==
  data: t input; u output; x input; tgrid input; xref input; K1flat input; K2grid input; unom input
function u = Gain_Selector(t, x, tgrid, xref, K1flat, K2grid, unom)
%#codegen
% Fixed-size output: u is always 4x1

u = zeros(4,1);

x = x(:);              % should be 13x1 for 6DOF
N = length(tgrid);

% --- Clamp time and compute interval index ---
if t <= tgrid(1)
    idx = 1;
    w = 0.0;
elseif t >= tgrid(end)
    idx = N-1;
    w = 1.0;
else
    idx = 1;
    for k = 1:(N-1)
        if tgrid(k) <= t && t < tgrid(k+1)
            idx = k;
            break;
        end
    end
    t1 = tgrid(idx);
    t2 = tgrid(idx+1);
    w  = (t - t1) / (t2 - t1);
end

% --- Interpolate reference state (13x1) ---
xref_t = (1-w)*xref(idx,:)' + w*xref(idx+1,:)';

% --- Interpolate K1flat then reshape to 4x13 ---
Kflat = (1-w)*K1flat(idx,:) + w*K1flat(idx+1,:);
K1 = reshape(Kflat, 13, 4)';   % 4x13   (requires K1flat is N×52)

% --- Interpolate K2 (4x1) ---
K2 = (1-w)*K2grid(idx,:)' + w*K2grid(idx+1,:)';

% --- Interpolate nominal control (4x1) ---
u_nom = (1-w)*unom(idx,:)' + w*unom(idx+1,:)';

q     = x(10:13);
qref  = xref_t(10:13);

if dot(q,qref) < 0
    q = -q;
end

x_used = x;
x_used(10:13) = q;

dx = x_used - xref_t;


% --- Control law ---
%dx = (x - xref_t);          % 13x1
u  =u_nom+(-K1*dx)-K2;  
%fix

end

== matlab function hopper_6dof_NED_v2_fluid_integration/Fluid Network2/Fuel Throttle Valve Controller/System ==
  data: Ptank input; CdA input; mdot input; Pout output; rho input; dp output
function [Pout,dp] = theta_to_pressure(Ptank,CdA,mdot, rho)

% CdA = mdot/(sqrt((2*(ptank-pout)*rho)

%CdA = max(CdA, 1e-7);
dp = (mdot/CdA)^2*1/(2*rho);

% (mdot/CdA)^2*rho/2 is solving for the pout from the dp in CdA eqn
Pout = Ptank - dp;
Pout = max(Pout, 0);

== matlab function hopper_6dof_NED_v2_fluid_integration/Fluid Network2/Injector1/Fuel Injector Calculations ==
  data: P_down input; rho input; mdot input; CdA input; stiffness output; P_up output; dP_inj output
function [stiffness, P_up, dP_inj] = injectorModel(P_down, rho, mdot, CdA)
%#codegen
% Injector model using known downstream pressure, density, mdot, and CdA
%
% Inputs:
%   P_down - Downstream / chamber pressure [Pa]
%   rho    - Fluid density [kg/m^3]
%   mdot   - Mass flow rate through injector [kg/s]
%   CdA    - Effective injector area, Cd*A [m^2]
%
% Outputs:
%   stiffness - Injector stiffness, S = dP_inj / P_down [-]
%   P_up      - Required upstream / manifold pressure [Pa]
%   dP_inj    - Pressure drop across injector [Pa]
%
% Equations:
%   mdot   = CdA * sqrt(2 * rho * dP_inj)
%   => dP_inj = (mdot / CdA)^2 / (2*rho)
%
%   P_up = P_down + dP_inj
%   stiffness = dP_inj / P_down

    % Compute pressure drop from orifice equation
    dP_inj = (mdot / CdA)^2 / (2 * rho);

    % Upstream pressure
    P_up = P_down + dP_inj;

    % Stiffness
    stiffness = dP_inj / P_down;

end

== matlab function hopper_6dof_NED_v2_fluid_integration/Fluid Network2/Injector2/Ox Injector Calculations ==
  data: P_down input; rho input; mdot input; CdA input; stiffness output; P_up output; dP_inj output
function [stiffness, P_up, dP_inj] = injectorModel(P_down, rho, mdot, CdA)
%#codegen
% Injector model using known downstream pressure, density, mdot, and CdA
%
% Inputs:
%   P_down - Downstream / chamber pressure [Pa]
%   rho    - Fluid density [kg/m^3]
%   mdot   - Mass flow rate through injector [kg/s]
%   CdA    - Effective injector area, Cd*A [m^2]
%
% Outputs:
%   stiffness - Injector stiffness, S = dP_inj / P_down [-]
%   P_up      - Required upstream / manifold pressure [Pa]
%   dP_inj    - Pressure drop across injector [Pa]
%
% Equations:
%   mdot   = CdA * sqrt(2 * rho * dP_inj)
%   => dP_inj = (mdot / CdA)^2 / (2*rho)
%
%   P_up = P_down + dP_inj
%   stiffness = dP_inj / P_down

    % Compute pressure drop from orifice equation
    dP_inj = (mdot / CdA)^2 / (2 * rho);

    % Upstream pressure
    P_up = P_down + dP_inj;

    % Stiffness
    stiffness = dP_inj / P_down;

end

== matlab function hopper_6dof_NED_v2_fluid_integration/Fluid Network2/MATLAB Function ==
  data: mdot_ox input; mdot_fuel input; eta_cstar input; Cf input; thrust output; Pc output; MR output; cstar_ideal input; mdot output
function [thrust, Pc, MR, mdot] = engine_model(mdot_ox, mdot_fuel, eta_cstar, Cf, cstar_ideal)
%#codegen
% ENGINE_MODEL
%
% Inputs:
%   mdot_ox      - oxidizer mass flow rate [kg/s]
%   mdot_fuel    - fuel mass flow rate [kg/s]
%   eta_cstar    - c* efficiency [-]
%   Cf           - thrust coefficient [-]
%
% Outputs:
%   thrust       - thrust [N]
%   Pc           - chamber pressure [Pa]
%   MR           - mixture ratio [-]

    %% -------------------------
    % CONSTANTS
    % -------------------------
    At = 0.0008271;      % throat area [m^2]

    %% -------------------------
    % 1. Total mass flow
    % -------------------------
    mdot = mdot_ox + mdot_fuel;

    %% -------------------------
    % 2. Mixture ratio
    % -------------------------
    if mdot_fuel > 0
        MR = mdot_ox / mdot_fuel;
    else
        MR = 0; % avoid divide by zero
    end

    %% -------------------------
    % 3. Actual c*
    % -------------------------
    cstar_actual = eta_cstar * cstar_ideal;

    %% -------------------------
    % 4. Chamber pressure
    % -------------------------
    Pc = (mdot * cstar_actual) / At;

    %% -------------------------
    % 6. Thrust
    % -------------------------
    thrust = Cf * Pc * At;

    % Equivalent:
    % thrust = Cf * mdot * cstar_actual;

end

== matlab function hopper_6dof_NED_v2_fluid_integration/Fluid Network2/Ox Throttle Valve Controller/Feed Forward ==
  data: mdot input; theta output; ptank input; pset input; rho input; CdA output
function [theta, CdA] = feed_forward(mdot,ptank,pset,rho)

dp = max(ptank - pset, 1e-6); % divide by zero erro

rho = max(rho, 1e-6);
CdA = mdot / sqrt(2*dp*rho);

CdA = max(CdA, 1e-7); % divide by zero error
Cv_vector = [1e-8, 0.01, 0.06, 0.21, 0.46, 0.83, 1.35, 2.04, 2.93];
CdA_vector = Cv_vector ./ 37.97;
theta_vector = 0.9.*[20,30,40,50,60,70,80,90,100];

theta = interp1(CdA_vector, theta_vector, CdA);
theta = min(theta, 90);
theta = max(theta, 0);
end

== matlab function hopper_6dof_NED_v2_fluid_integration/Fluid Network2/Ox Throttle Valve Controller/MATLAB Function5 ==
  data: time input; rate_limit_up output; rate_limit_down output
function [rate_limit_up, rate_limit_down] = fcn(time)
if time < 0.5
    rate_limit_up = 1350;
else
    rate_limit_up = 40;
end
rate_limit_down = -rate_limit_up;

== matlab function hopper_6dof_NED_v2_fluid_integration/Fluid Network2/Ox Throttle Valve Controller/System ==
  data: Ptank input; CdA input; mdot input; Pout output; rho input; dp output
function [Pout,dp] = theta_to_pressure(Ptank,CdA,mdot, rho)

% CdA = mdot/(sqrt((2*(ptank-pout)*rho)

%CdA = max(CdA, 1e-7);
dp = (mdot/CdA)^2*1/(2*rho);

% (mdot/CdA)^2*rho/2 is solving for the pout from the dp in CdA eqn
Pout = Ptank - dp;
Pout = max(Pout, 0);

== matlab function hopper_6dof_NED_v2_fluid_integration/Fluid Network2/Thrust Commanded to mdot + bunch of other bs ==
  data: mdot_fuel output; rho_fuel_eng output; pc output; F_cmd input; rho_ox input; rho_fuel input; rho_ox_eng output; mdot_ox output; Cf input; MR input; cstar_ideal input; cstar_eff input
function [mdot_fuel, rho_fuel_eng, pc, rho_ox_eng, mdot_ox] = thrust_to_mdot( ...
   F_cmd, rho_ox, rho_fuel, Cf, MR, cstar_ideal, cstar_eff)
%#codegen
% Convert commanded thrust into mdots and convert densities to English units
%
% Outputs:
%   mdot_ox        - oxidizer mass flow rate [kg/s]
%   mdot_fuel      - fuel mass flow rate [kg/s]
%   rho_ox_eng     - oxidizer density [lb/ft^3]
%   rho_fuel_eng   - fuel density [lb/ft^3]
%   mdot_ox_lb     - oxidizer mass flow rate [lb/s]
%   mdot_fuel_lb   - fuel mass flow rate [lb/s]

    cstar = cstar_ideal * cstar_eff;
    At = 0.0008271;      % throat area [m^2]

    %% ---- DEFAULT OUTPUTS ----
    mdot_ox = 0;
    mdot_fuel = 0;
    rho_ox_eng = 0;
    rho_fuel_eng = 0;
    mdot_ox_lb = 0;
    mdot_fuel_lb = 0;

    %% ---- UNIT CONVERSION ----
    kgm3_to_lbft3 = 0.062428;
    kg_to_lb = 2.20462;

    rho_ox_eng = rho_ox * kgm3_to_lbft3;
    rho_fuel_eng = rho_fuel * kgm3_to_lbft3;

    %% ---- EFFECTIVE EXHAUST VELOCITY ----
    ve = Cf * cstar;


    %% ---- TOTAL MASS FLOW ----
    mdot_total = F_cmd / ve;

    pc = mdot_total * cstar / At;

    pc = pc * 0.000145038;

    %% ---- SPLIT BY MR ----
    mdot_ox = mdot_total * MR / (1 + MR);
    mdot_fuel = mdot_total / (1 + MR);


end

== matlab function hopper_6dof_NED_v2_fluid_integration/Ground_Contact/Inertial Leg Velocity/MATLAB Function ==
  data: a input; y output; b input
function y = crossProduct(a, b)
    y = cross(repmat(a,1,4), b, 1);

== matlab function hopper_6dof_NED_v2_fluid_integration/Ground_Contact/MATLAB Function ==
  data: a input; y output; b input
function y = crossProduct(a, b)
    y = cross(a, b);

== matlab function hopper_6dof_NED_v2_fluid_integration/Slosh/MATLAB Function1 ==
  data: fu_mass input; fu_lateral_natural_freq output; fu_axial_natural_freq output; fu_lateral_slosh_mass output; fu_aeff input; fu_axial_slosh_mass output; fu_lateral_pendulum_l output; fu_axial_pendulum_l output; fu_lateral_damping output; fu_axial_damping output; tank_r input; fu_lateral_damping input; fu_axial_damping input
function [fu_lateral_natural_freq, fu_axial_natural_freq, fu_lateral_slosh_mass,fu_axial_slosh_mass, fu_lateral_pendulum_l, fu_axial_pendulum_l, fu_lateral_damping, fu_axial_damping]  = slosh_parameters(fu_mass, fu_aeff, tank_r, fu_lateral_damping, fu_axial_damping)

% Flat-bottomed cylindrical tank, linear slosh (NASA SP-106 / Dodge 2000;
% lateral values checked against SLOSH-ML, lgst-lab/slosh_ml).
zeta = 1.841;    % 1st root of J1' (1st lateral mode)
eps01 = 3.8317;  % 1st root of J1 (1st axisymmetric mode)
fu_density = 800;   % kg/m^3
geff = norm(fu_aeff) + 0.001;

if fu_mass > 0.001
   h_fu_fluid = (fu_mass / fu_density) / (pi * tank_r^2);

   % Lateral mode: omega^2 = (g*xi/R) * tanh(xi*h/R)
    fu_lateral_natural_freq = sqrt(zeta * geff / tank_r * tanh(zeta * h_fu_fluid / tank_r));
    fu_lateral_slosh_mass = fu_mass * (2 * tank_r * tanh(zeta * h_fu_fluid / tank_r)) / (zeta * (zeta^2 - 1) * h_fu_fluid);
    fu_lateral_pendulum_l = tank_r / (zeta * tanh(zeta * h_fu_fluid / tank_r));   % = geff / omega^2

    % Axisymmetric (m = 0) mode: omega^2 = (g*eps01/R) * tanh(eps01*h/R).
    % Volume is conserved and the mode is axisymmetric, so to first order
    % it puts no net force or moment on the tank: its equivalent mechanical
    % mass is zero. The oscillator is kept (frequency/damping) but couples
    % no force or roll torque into the vehicle.
    fu_axial_natural_freq = sqrt(eps01 * geff / tank_r * tanh(eps01 * h_fu_fluid / tank_r));
    fu_axial_slosh_mass = 0;
    fu_axial_pendulum_l = geff / fu_axial_natural_freq^2;
else
   h_fu_fluid = 0;
   fu_lateral_natural_freq = 0;
   fu_axial_natural_freq = 0;
   fu_lateral_slosh_mass = 0;
   fu_axial_slosh_mass = 0;
   fu_lateral_pendulum_l = 1;
   fu_axial_pendulum_l = 1;
end

end

== matlab function hopper_6dof_NED_v2_fluid_integration/Slosh/Oxidizer Pitch Force/MATLAB Function ==
  data: ox_pitch_accel input; accel_term output; ox_lateral_pendulum_l input
function accel_term = fcn(ox_pitch_accel, ox_lateral_pendulum_l)

accel_term = -ox_pitch_accel / ox_lateral_pendulum_l;

end

== matlab function hopper_6dof_NED_v2_fluid_integration/Slosh/Oxidizer Pitch Force/MATLAB Function1 ==
  data: ox_pitch_phi input; ang_term output; ox_lateral_natural_freq input
function ang_term = fcn(ox_pitch_phi, ox_lateral_natural_freq)

ang_term = -ox_lateral_natural_freq^2 * ox_pitch_phi;

end

== matlab function hopper_6dof_NED_v2_fluid_integration/Slosh/Oxidizer Pitch Force/MATLAB Function2 ==
  data: ox_pitch_phi_dot input; velo_term output; ox_lateral_natural_freq input; ox_lateral_damping input
function velo_term = fcn(ox_pitch_phi_dot, ox_lateral_natural_freq,ox_lateral_damping)

velo_term = -2 * ox_lateral_damping * ox_lateral_natural_freq * ox_pitch_phi_dot;
end

== matlab function hopper_6dof_NED_v2_fluid_integration/Slosh/Oxidizer Pitch Force/MATLAB Function3 ==
  data: ox_pitch_phi_ddot input; ox_pitch_f output; ox_lateral_slosh_mass input; ox_lateral_pendulum_l input
function ox_pitch_f = fcn(ox_pitch_phi_ddot, ox_lateral_slosh_mass, ox_lateral_pendulum_l)
% Force of the pendulum on the tank, beyond the rigid propellant already in
% the vehicle mass: -m1 * y_ddot, y = l*phi the body-frame bob displacement
% (phi_ddot = -a/l - w^2 phi - 2 zeta w phi_dot). Sign was +m1*y_ddot,
% which added m1 to the lateral inertia instead of removing it.
ox_pitch_f = -ox_lateral_slosh_mass * ox_lateral_pendulum_l * ox_pitch_phi_ddot;
end
